simulink model "conference_model"  (R2022b)
settings: Solver=VariableStepAuto  StartTime=0  StopTime=0.7  RelTol=1e-3
undefined symbols (not defined in the file): Iabc1, Iabc2, Iabc3, Vabc1, Vabc2, Vabc3
libraries: spsThreePhasePISectionLineLib x6, spsThreePhaseFaultLib x3, spsThreePhaseSeriesRLCLoadLib x3, spsThreePhaseVIMeasurementLib x3, spsThreePhaseSourceLib x2, spspowerguiLib x1
settings Model: Creator=AURONNO  LastModifiedBy=DELL
settings SolverCC: AlgebraicLoopSolver=TrustRegion
settings DebuggingCC: UnconnectedInputMsg=warning  UnconnectedOutputMsg=warning  UnconnectedLineMsg=warning  SFMachineParentedDataDiag=warning
settings ModelReferenceCC: EnableRefExpFcnMdlSchedulingChecks=on
settings RTWCC: DLArmComputeVersion=19.05

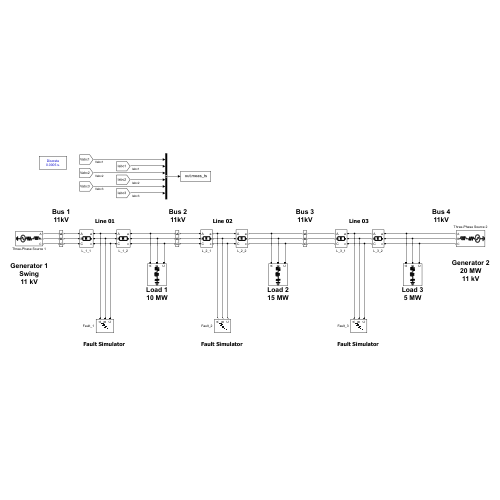
[thumbnail: Simulink's stored preview of the top-level diagram]
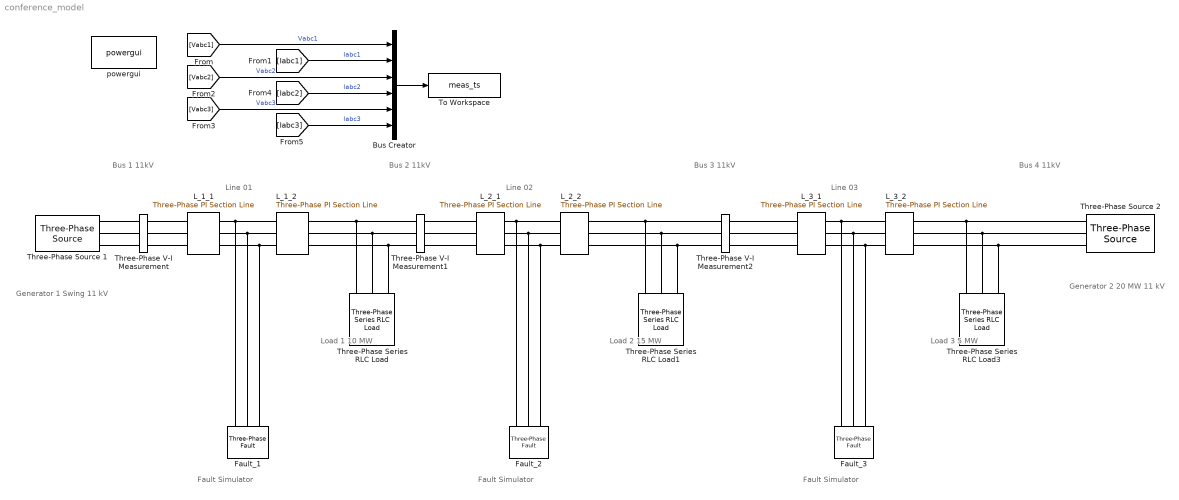
== system conference_model ==
  note: Line 01
  note: Bus 1
      | 11kV
  note: Bus 2
      | 11kV
  note: Bus 3
      | 11kV
  note: Bus 4
      | 11kV
  note: Generator 1
      | Swing
      | 11 kV
  note: Generator 2
      | 20 MW
      | 11 kV
  note: Load 1
      | 10 MW
  note: Load 2
      | 15 MW
  note: Load 3
      | 5 MW
  note: Line 02
  note: Line 03
  note: Fault Simulator
  note: Fault Simulator
  note: Fault Simulator
  Bus Creator : BusCreator  Inputs=Vabc1,Iabc1,Vabc2,Iabc2,Vabc3,Iabc3
  Fault_1 : spsThreePhaseFaultLib/Three-Phase Fault  InitialStates=0  FaultA=off  FaultB=off  FaultC=off  GroundFault=off  SwitchTimes=[0.25 0.65]  External=off  SwitchStatus=NaN  FaultResistance=5  GroundResistance=0.01  SnubberResistance=1e6  SnubberCapacitance=inf  Measurements=Fault voltages and currents
  Fault_2 : spsThreePhaseFaultLib/Three-Phase Fault  InitialStates=0  FaultA=off  FaultB=off  FaultC=off  GroundFault=off  SwitchTimes=[0.09 0.11]  External=off  SwitchStatus=NaN  FaultResistance=10  GroundResistance=0.01  SnubberResistance=1e6  SnubberCapacitance=inf  Measurements=None
  Fault_3 : spsThreePhaseFaultLib/Three-Phase Fault  InitialStates=0  FaultA=off  FaultB=off  FaultC=off  GroundFault=off  SwitchTimes=[0.13 0.15]  External=off  SwitchStatus=NaN  FaultResistance=10  GroundResistance=0.01  SnubberResistance=1e6  SnubberCapacitance=inf  Measurements=None
  L_1_1 : spsThreePhasePISectionLineLib/Three-Phase PI Section Line  LConnTagsString=a|b|c  RConnTagsString=A|B|C  Length=2  Frequency=50  Resistances=[0.044965 0.11241]  Inductances="[ 1.414e-3  3.53e-3]"  Capacitances=[10.47e-9 6.15e-9]
  L_1_2 : spsThreePhasePISectionLineLib/Three-Phase PI Section Line  LConnTagsString=a|b|c  RConnTagsString=A|B|C  Length=98  Frequency=50  Resistances=[0.044965 0.11241]  Inductances="[ 1.414e-3  3.53e-3]"  Capacitances=[10.47e-9 6.15e-9]
  L_2_1 : spsThreePhasePISectionLineLib/Three-Phase PI Section Line  LConnTagsString=a|b|c  RConnTagsString=A|B|C  Length=50  Frequency=50  Resistances=[0.044965 0.11241]  Inductances="[ 1.414e-3  3.53e-3]"  Capacitances=[10.47e-9 6.15e-9]
  L_2_2 : spsThreePhasePISectionLineLib/Three-Phase PI Section Line  LConnTagsString=a|b|c  RConnTagsString=A|B|C  Length=50  Frequency=50  Resistances=[0.044965 0.11241]  Inductances="[ 1.414e-3  3.53e-3]"  Capacitances=[10.47e-9 6.15e-9]
  L_3_1 : spsThreePhasePISectionLineLib/Three-Phase PI Section Line  LConnTagsString=a|b|c  RConnTagsString=A|B|C  Length=50  Frequency=50  Resistances=[0.044965 0.11241]  Inductances="[ 1.414e-3  3.53e-3]"  Capacitances=[10.47e-9 6.15e-9]
  L_3_2 : spsThreePhasePISectionLineLib/Three-Phase PI Section Line  LConnTagsString=a|b|c  RConnTagsString=A|B|C  Length=50  Frequency=50  Resistances=[0.044965 0.11241]  Inductances="[ 1.414e-3  3.53e-3]"  Capacitances=[10.47e-9 6.15e-9]
  Three-Phase Series RLC Load : spsThreePhaseSeriesRLCLoadLib/Three-Phase Series RLC Load  LConnTagsString=A|B|C  Configuration=Y (grounded)  NominalVoltage=11e3  Vabc=[1e3 1e3 1e3]  Vabcp=[1e3 1e3 1e3]  NominalFrequency=50  UnbalancedPower=off  ActivePower=10e6  InductivePower=3e6  CapacitivePower=100  Pabc=[10e3 9e3 11e3]  QLabc=[100 90 110]  QCabc=[100 90 110]  Pabcp=[10e3 9e3 11e3]  QLabcp=[100 90 110]  QCabcp=[100 90 110]  Measurements=Branch voltages and currents  LoadType=constant PQ
  Three-Phase Series RLC Load1 : spsThreePhaseSeriesRLCLoadLib/Three-Phase Series RLC Load  LConnTagsString=A|B|C  Configuration=Y (grounded)  NominalVoltage=11e3  Vabc=[1e3 1e3 1e3]  Vabcp=[1e3 1e3 1e3]  NominalFrequency=50  UnbalancedPower=off  ActivePower=15e6  InductivePower=2e6  CapacitivePower=100  Pabc=[10e3 9e3 11e3]  QLabc=[100 90 110]  QCabc=[100 90 110]  Pabcp=[10e3 9e3 11e3]  QLabcp=[100 90 110]  QCabcp=[100 90 110]  Measurements=Branch voltages and currents  LoadType=constant PQ
  Three-Phase Series RLC Load3 : spsThreePhaseSeriesRLCLoadLib/Three-Phase Series RLC Load  LConnTagsString=A|B|C  Configuration=Y (grounded)  NominalVoltage=11e3  Vabc=[1e3 1e3 1e3]  Vabcp=[1e3 1e3 1e3]  NominalFrequency=50  UnbalancedPower=off  ActivePower=5e6  InductivePower=1e6  CapacitivePower=100  Pabc=[10e3 9e3 11e3]  QLabc=[100 90 110]  QCabc=[100 90 110]  Pabcp=[10e3 9e3 11e3]  QLabcp=[100 90 110]  QCabcp=[100 90 110]  Measurements=Branch voltages and currents  LoadType=constant PQ
  Three-Phase V-I Measurement : spsThreePhaseVIMeasurementLib/Three-Phase V-I Measurement  VoltageMeasurement=phase-to-ground  SetLabelV=on  LabelV=Vabc1  Vpu=off  VpuLL=off  CurrentMeasurement=yes  SetLabelI=on  LabelI=Iabc1  Ipu=off  Pbase=100e6  Vbase=500e3  OutputType=Complex  PhasorSimulation=off  PSBequivalent=0
  Three-Phase V-I Measurement1 : spsThreePhaseVIMeasurementLib/Three-Phase V-I Measurement  VoltageMeasurement=phase-to-ground  SetLabelV=on  LabelV=Vabc2  Vpu=off  VpuLL=off  CurrentMeasurement=yes  SetLabelI=on  LabelI=Iabc2  Ipu=off  Pbase=100e6  Vbase=500e3  OutputType=Complex  PhasorSimulation=off  PSBequivalent=0
  Three-Phase V-I Measurement2 : spsThreePhaseVIMeasurementLib/Three-Phase V-I Measurement  VoltageMeasurement=phase-to-ground  SetLabelV=on  LabelV=Vabc3  Vpu=off  VpuLL=off  CurrentMeasurement=yes  SetLabelI=on  LabelI=Iabc3  Ipu=off  Pbase=100e6  Vbase=500e3  OutputType=Complex  PhasorSimulation=off  PSBequivalent=0
  Three-Phase Source 1 : spsThreePhaseSourceLib/Three-Phase Source  InternalConnection=Yg  VoltagePhases=off  Voltage=11e3  PhaseAngle=0  Voltage_phases=[25e3 25e3 25e3]/sqrt(3)  PhaseAngles_phases=[0 -120 +120]  Frequency=50  NonIdealSource=on  SpecifyImpedance=off  Resistance=0.8929  Inductance=16.58e-3  ShortCircuitLevel=100e6  BaseVoltage=11e3  XRratio=7  BusType=swing  Pref=100e6  Qref=0  Prefabc=[10e3, 10e3, 10e3]  Qrefabc=[0, 0, 0]  Qmin=-inf  Qmax=inf
  Three-Phase Source 2 : spsThreePhaseSourceLib/Three-Phase Source  InternalConnection=Yg  VoltagePhases=off  Voltage=11e3  PhaseAngle=0  Voltage_phases=[25e3 25e3 25e3]/sqrt(3)  PhaseAngles_phases=[0 -120 +120]  Frequency=50  NonIdealSource=on  SpecifyImpedance=off  Resistance=0.8929  Inductance=16.58e-3  ShortCircuitLevel=100e6  BaseVoltage=11e3  XRratio=7  BusType=PV  Pref=20e6  Qref=0  Prefabc=[10e3, 10e3, 10e3]  Qrefabc=[0, 0, 0]  Qmin=-inf  Qmax=inf
  To Workspace : ToWorkspace  VariableName=meas_ts  SaveFormat=Timeseries  SampleTime=-1
  powergui : spspowerguiLib/powergui  Priority=1  SimulationMode=Discrete  SampleTime=500e-6  frequency=60  Iterations=50  frequencyindice=50  Pbase=100e6  ErrMax=1e-4  UnitsV=kV  UnitsW=MW  buscounter=0  FunctionMessages=off  echomessages=off  EnableUseOfTLC=off  CurrentSourceSwitches=off  DisableSnubberDevices=off  DisableRonSwitches=off  DisableVfSwitches=off  DisplayEquations=off  AutomaticDiscreteSolvers=off  SolverType=Tustin/Backward Euler (TBE)  Interpol=off  ExternalGateDelay=off  methode=off  Ts=100  x0status=blocks  SPID=on  SwTol=0  HookPort=off  NonlinearTolerance=1e-4  nMaxIteration=100  ContinueOnMaxIteration=off  RestoreLinks=warning  ResistiveCurrentMeasurement=off  Frange=[0:2:500]  Ylog=off  Xlog=on  ShowGrid=off  save=off  variable=ZData  structure=0  ZoomFFT=off  StartTime=0.0  cycles=1  DisplayStyle=1  fundamental=60  FreqAxis=off  MaxFrequency=1000  frequencyindicesteady=1  RmsSteady=1  display=off
  wires:
  Bus Creator/1 -> To Workspace/1
  [Vabc2] -> Bus Creator/3  "Vabc2"
  [Vabc3] -> Bus Creator/5  "Vabc3"
  [Iabc2] -> Bus Creator/4  "Iabc2"
  [Iabc3] -> Bus Creator/6  "Iabc3"
  [Vabc1] -> Bus Creator/1  "Vabc1"
  [Iabc1] -> Bus Creator/2  "Iabc1"
  connections:
  Three-Phase Source 1/RConn1 -- Three-Phase V-I Measurement/LConn1
  Three-Phase Source 1/RConn2 -- Three-Phase V-I Measurement/LConn2
  Three-Phase Source 1/RConn3 -- Three-Phase V-I Measurement/LConn3
  Three-Phase V-I Measurement/RConn1 -- L_1_1/LConn1
  Three-Phase V-I Measurement/RConn2 -- L_1_1/LConn2
  Three-Phase V-I Measurement/RConn3 -- L_1_1/LConn3
  L_1_1/RConn1 -- L_1_2/LConn1 -- Fault_1/LConn1
  L_1_1/RConn2 -- L_1_2/LConn2 -- Fault_1/LConn2
  L_1_1/RConn3 -- L_1_2/LConn3 -- Fault_1/LConn3
  Three-Phase Series RLC Load/LConn1 -- Three-Phase V-I Measurement1/LConn1 -- L_1_2/RConn1
  Three-Phase Series RLC Load/LConn2 -- Three-Phase V-I Measurement1/LConn2 -- L_1_2/RConn2
  L_1_2/RConn3 -- Three-Phase V-I Measurement1/LConn3 -- Three-Phase Series RLC Load/LConn3
  L_2_2/LConn1 -- Fault_2/LConn1 -- L_2_1/RConn1
  L_2_1/RConn2 -- L_2_2/LConn2 -- Fault_2/LConn2
  L_2_1/RConn3 -- L_2_2/LConn3 -- Fault_2/LConn3
  L_2_2/RConn3 -- Three-Phase V-I Measurement2/LConn3 -- Three-Phase Series RLC Load1/LConn3
  Three-Phase Series RLC Load1/LConn1 -- Three-Phase V-I Measurement2/LConn1 -- L_2_2/RConn1
  Three-Phase Series RLC Load1/LConn2 -- Three-Phase V-I Measurement2/LConn2 -- L_2_2/RConn2
  L_3_1/RConn3 -- L_3_2/LConn3 -- Fault_3/LConn3
  L_3_1/RConn2 -- L_3_2/LConn2 -- Fault_3/LConn2
  L_3_1/RConn1 -- Fault_3/LConn1 -- L_3_2/LConn1
  Three-Phase V-I Measurement1/RConn1 -- L_2_1/LConn1
  Three-Phase V-I Measurement1/RConn2 -- L_2_1/LConn2
  Three-Phase V-I Measurement1/RConn3 -- L_2_1/LConn3
  Three-Phase V-I Measurement2/RConn1 -- L_3_1/LConn1
  Three-Phase V-I Measurement2/RConn2 -- L_3_1/LConn2
  Three-Phase V-I Measurement2/RConn3 -- L_3_1/LConn3
  L_3_2/RConn1 -- Three-Phase Source 2/RConn1 -- Three-Phase Series RLC Load3/LConn1
  Three-Phase Series RLC Load3/LConn2 -- Three-Phase Source 2/RConn2 -- L_3_2/RConn2
  L_3_2/RConn3 -- Three-Phase Source 2/RConn3 -- Three-Phase Series RLC Load3/LConn3
